simulink model "SMC_PTC"  (R2026b)
settings Model: Creator=nesti  LastModifiedBy=Yahoff

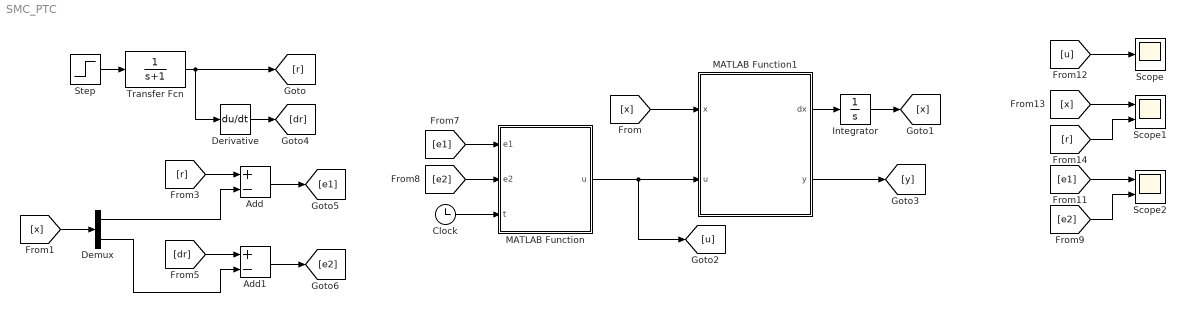
== system SMC_PTC ==
  Add : Sum  Inputs=+-
  Add1 : Sum  Inputs=+-
  Clock : Clock
  Demux : Demux  Outputs=2
  Derivative : Derivative
  Integrator : Integrator  InitialCondition=3
  MATLAB Function : MATLAB Function  TreatAsAtomicUnit=on
  MATLAB Function1 : MATLAB Function  TreatAsAtomicUnit=on
  Scope : Scope
      settings: ActiveDisplayYMinimum=-86.664974626828567  ActiveDisplayYMaximum=38.784771641457105
  Scope1 : Scope  NumInputPorts=2
      settings: ActiveDisplayYMinimum=-0.625020528829724  ActiveDisplayYMaximum=5.6251847594675173
  Scope2 : Scope  NumInputPorts=2
      settings: ActiveDisplayYMinimum=-4.25  ActiveDisplayYMaximum=8.25  DataLoggingVariableName=ScopeData2
  Step : Step  Time=0  FinalValue=5  SampleTime=0
  Transfer Fcn : TransferFcn  Denominator=[1 1]
  wires:
  Step/1 -> Transfer Fcn/1
  Transfer Fcn/1 -> Derivative/1, [r]
  MATLAB Function1/1(dx) -> Integrator/1
  Integrator/1 -> [x]
  [x] -> MATLAB Function1/1(x)
  MATLAB Function/1(u) -> [u], MATLAB Function1/2(u)
  Derivative/1 -> [dr]
  [r] -> Add/1
  Demux/1 -> Add/2
  Add/1 -> [e1]
  Add1/1 -> [e2]
  Demux/2 -> Add1/2
  [dr] -> Add1/1
  [e1] -> MATLAB Function/1(e1)
  [e2] -> MATLAB Function/2(e2)
  Clock/1 -> MATLAB Function/3(t)
  [u] -> Scope/1
  [x] -> Scope1/1
  [r] -> Scope1/2
  [e1] -> Scope2/1
  [e2] -> Scope2/2
  MATLAB Function1/2(y) -> [y]
  [x] -> Demux/1

== matlab function SMC_PTC/MATLAB Function1 ==
  data: x input size=2; dx output size=2; u input; y output
function [dx, y]= planta(x , u)

x1 = x(1);
x2 = x(2);

dx1 = x2;
dx2 = sin(x1+x2) + u;
y = x1;

dx = [dx1;dx2];

== matlab function SMC_PTC/MATLAB Function ==
  data: u output; e1 input; e2 input; t input
function u  = controlador(e1, e2, t)


T = 5; 
m = 10;
K = 25;

% r(0)=0, dr(0)=0
a = -3; % x1(0)=3
b = 2; % x2(0)=-2

% Coeficientes
c = 2*a + b*T;
tau = t/T;

% Trayectorias auxiliares
if t < T

    e1a = (1-tau)^2*(a+c*tau);

    e2a = b - (2/T)*(3*a+2*b*T)*tau ...
        + (3*c/T)*tau^2;

    dde1a = -(2/T^2)*(3*a+2*b*T) ...
        + (6*c/T^2)*tau;

else

    e1a = 0;
    e2a = 0;
    dde1a = 0;

end

eps1 = e1a - e1;
eps2 = e2a - e2;

s = eps2 + m*eps1;

u = -dde1a - m*eps2 - K*sign(s);
